simulink model "Lab1_3_2_3_RobustErrorSpc"  (R2024b)
settings: Solver=ode5  StartTime=0.0  StopTime=10  FixedStep=1e-03  RelTol=1e-3
undefined symbols (not defined in the file): alpha, degs2rpm, delta_i, k_ksi, km, National_Instruments, PCI, rpm2rads, sens, w0, wc, wc2
libraries: sldrtlib x2
settings Model: SimulationMode=external  ExtModeTrigDuration=45001  Creator=lenovo  LastModifiedBy=aboulenien
settings DataIOCC: ReturnWorkspaceOutputs=off
settings HardwareCC: ProdBitPerLong=64  ProdHWDeviceType=Intel->x86-64 (Linux 64)
settings RTWCC: Description=Simulink Desktop Real-Time  SystemTargetFile=sldrt.tlc  TemplateMakefile=sldrt.tmf  RTWCompilerOptimization=on
settings CodeAppCC: MaxIdLength=95
settings SimulinkDesktopRealTimeCC: TargetLibSuffix=_sldrt.a  TargetPreCompLibLocation=C:\Program Files\MATLAB\R2024b\toolbox\sldrt\lib\win64  ParMdlRefBuildCompliant=on

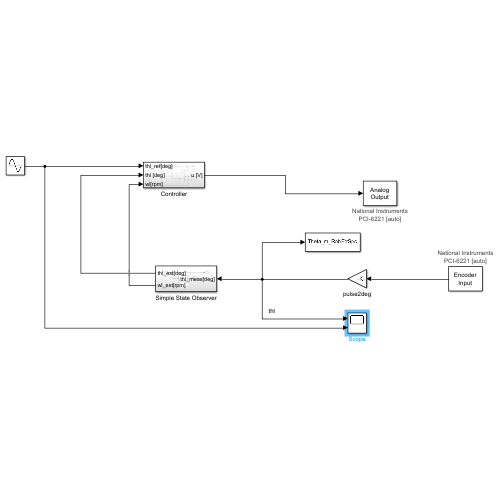
[thumbnail: Simulink's stored preview of the top-level diagram]
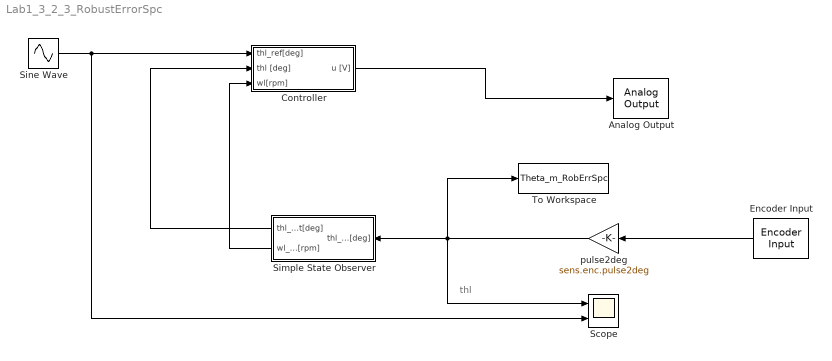
== system Lab1_3_2_3_RobustErrorSpc ==
  note: thl
  Analog Output : sldrtlib/Analog Output  SampleTime=-1  MaxMissedTicks=10  ShowMissedTicks=off  YieldWhenWaiting=off  DrvName=National_Instruments/PCI-6221  DrvAddress=4294967295  DrvOptions=[0 0 0 2 0]  Channels=1  RangeMode=1  VoltRange=1  InitialValue=0  FinalValue=0
      settings: AttributesFormatString=National Instruments\nPCI-6221 [auto]
  Controller : Subsystem
  Encoder Input : sldrtlib/Encoder Input  SampleTime=-1  MaxMissedTicks=10  ShowMissedTicks=off  YieldWhenWaiting=off  DrvName=National_Instruments/PCI-6221  DrvAddress=4294967295  DrvOptions=[0 0 0 2 0]  Channels=1  QuadMode=3  IndexPulse=1  InputFilter=Inf  DataType=1
      settings: AttributesFormatString=National Instruments\nPCI-6221 [auto]
  Scope : Scope  NumInputPorts=2
  Simple State Observer : Subsystem
  Sine Wave : Sin  Amplitude=90  Frequency=w0  SampleTime=0
  To Workspace : ToWorkspace  VariableName=Theta_m_RobErrSpc  SaveFormat=Structure With Time  SampleTime=0.001
  pulse2deg : Gain  Gain=sens.enc.pulse2deg
  wires:
  Encoder Input/1 -> pulse2deg/1
  pulse2deg/1 -> To Workspace/1, Scope/1, Simple State Observer/1(thl_meas[deg])
  Controller/1(u [V]) -> Analog Output/1
  Sine Wave/1 -> Scope/2, Controller/1(thl_ref[deg])
  Simple State Observer/1(thl_est[deg]) -> Controller/2(thl [deg])
  Simple State Observer/2(wl_est[rpm]) -> Controller/3(wl[rpm])

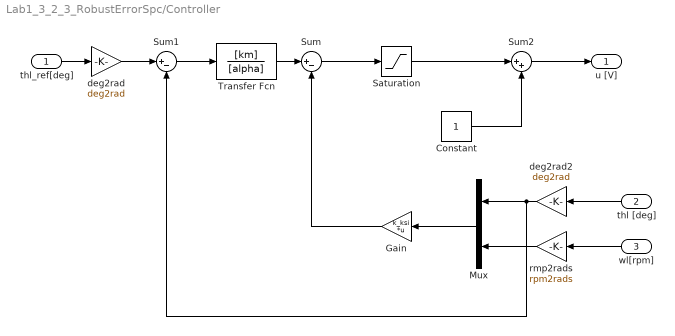
== system Lab1_3_2_3_RobustErrorSpc/Controller ==
  thl_ref[deg] : Inport
  thl [deg] : Inport  Port=2
  wl[rpm] : Inport  Port=3
  Constant : Constant
  Gain : Gain  Gain=k_ksi  Multiplication=Matrix(K*u)
  Mux : Mux  Inputs=2
  Saturation : Saturate  UpperLimit=12  LowerLimit=-12
  Sum : Sum  Inputs=|+-
  Sum1 : Sum  Inputs=|+-
  Sum2 : Sum  Inputs=|++
  Transfer Fcn : TransferFcn  Numerator=[km]  Denominator=[alpha]
  deg2rad : Gain  Gain=deg2rad
  deg2rad2 : Gain  Gain=deg2rad
  rmp2rads : Gain  Gain=rpm2rads
  u [V] : Outport
  wires:
  thl_ref[deg]/1 -> deg2rad/1
  deg2rad2/1 -> Mux/1, Sum1/2
  rmp2rads/1 -> Mux/2
  thl [deg]/1 -> deg2rad2/1
  wl[rpm]/1 -> rmp2rads/1
  Sum/1 -> Saturation/1
  Transfer Fcn/1 -> Sum/1
  Mux/1 -> Gain/1
  Gain/1 -> Sum/2
  deg2rad/1 -> Sum1/1
  Sum1/1 -> Transfer Fcn/1
  Constant/1 -> Sum2/2
  Saturation/1 -> Sum2/1
  Sum2/1 -> u [V]/1

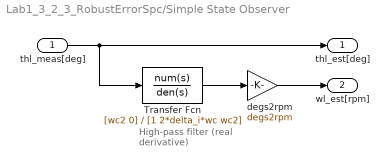
== system Lab1_3_2_3_RobustErrorSpc/Simple State Observer ==
  note: High-pass filter
      | (real derivative)
  thl_meas[deg] : Inport
  Transfer Fcn : TransferFcn  Numerator=[wc2 0]  Denominator=[1 2*delta_i*wc wc2]
  degs2rpm : Gain  Gain=degs2rpm
  thl_est[deg] : Outport
  wl_est[rpm] : Outport  Port=2
  wires:
  thl_meas[deg]/1 -> Transfer Fcn/1, thl_est[deg]/1
  Transfer Fcn/1 -> degs2rpm/1
  degs2rpm/1 -> wl_est[rpm]/1
